simulink model "simulare1"  (R2026a)
settings: Solver=FixedStepAuto  StopTime=0.5  FixedStep=1e-6
values from neighbouring files (symbols this model uses):
  C = delta_I_l/(8*fs*delta_U_out)    (= 0.0021875)    [proiect.m]    (also in tema3.m = 0.0018)
  C_real = 1800e-6    (= 0.0018)    [proiect.m]
  L = (u_in - u_out)*mu/(fs*delta_I_l)    (= 0.00260416666667)    [proiect.m]    (also in tema3.m = 0.0025)
  L_real = 2.5e-3    (= 0.0025)    [proiect.m]
  mu = u_out/u_in    (= 0.416666666667)    [proiect.m]    (also in tema2_simscape.m; tema3_figuri.m = out.logsout.get('mu').Values)
  R = u_out/I_out_max    (= 1.25)    [proiect.m]    (also in tema2_simscape.m; tema3.m)
settings Model: Creator=Fer Alexandru  LastModifiedBy=Fer Alexandru

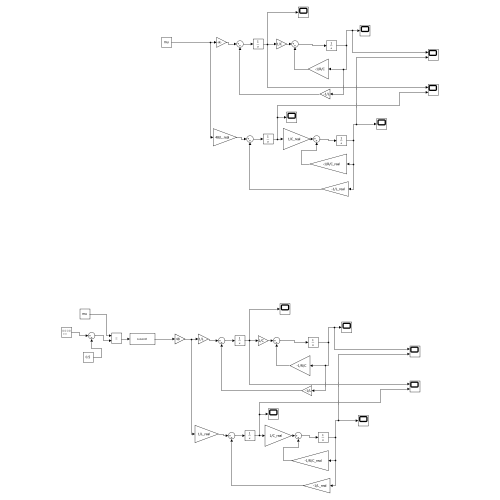
[thumbnail: Simulink's stored preview of the top-level diagram]
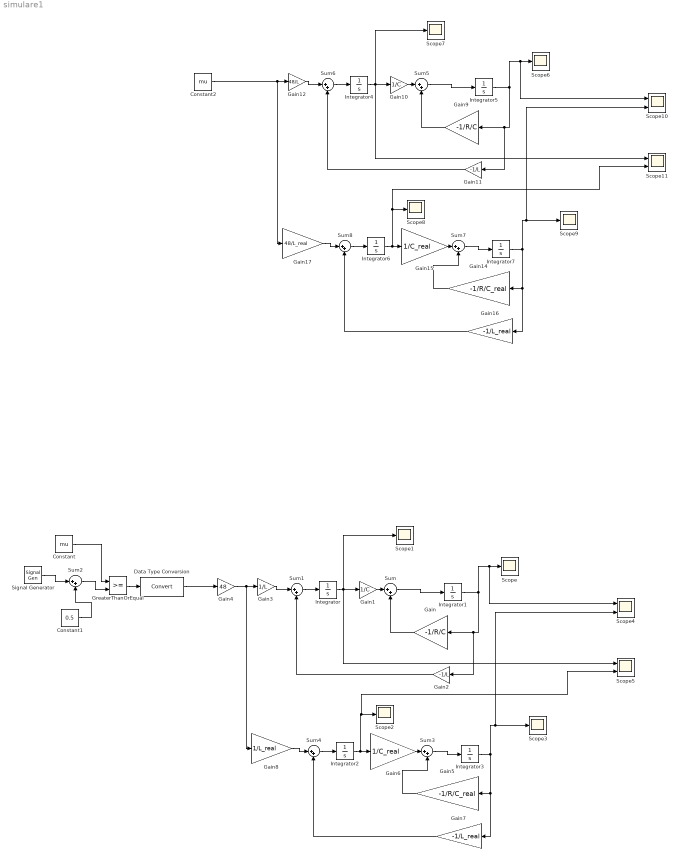
== system simulare1 ==
  Constant : Constant  Value=mu
  Constant1 : Constant  Value=0.5
  Constant2 : Constant  Value=mu
  Data Type Conversion : DataTypeConversion  SaturateOnIntegerOverflow=off  RndMeth=Floor
  Gain : Gain  Gain=-1/R/C
  Gain1 : Gain  Gain=1/C
  Gain10 : Gain  Gain=1/C
  Gain11 : Gain  Gain=-1/L
  Gain12 : Gain  Gain=48/L
  Gain14 : Gain  Gain=-1/R/C_real
  Gain15 : Gain  Gain=1/C_real
  Gain16 : Gain  Gain=-1/L_real
  Gain17 : Gain  Gain=48/L_real
  Gain2 : Gain  Gain=-1/L
  Gain3 : Gain  Gain=1/L
  Gain4 : Gain  Gain=48
  Gain5 : Gain  Gain=-1/R/C_real
  Gain6 : Gain  Gain=1/C_real
  Gain7 : Gain  Gain=-1/L_real
  Gain8 : Gain  Gain=1/L_real
  Gain9 : Gain  Gain=-1/R/C
  GreaterThanOrEqual : RelationalOperator  OutDataTypeStr=boolean  RndMeth=Simplest  InputSameDT=off
  Integrator{,1..7} (8 alike) : Integrator
  Scope{,1..3,6..9} (8 alike) : Scope
      Scope settings: ActiveDisplayYMinimum=19.471806262119504  ActiveDisplayYMaximum=19.914867992348224
      Scope1 settings: ActiveDisplayYMinimum=-2.4653855800406355  ActiveDisplayYMaximum=41.613009879574278
      Scope2 settings: ActiveDisplayYMinimum=38.565618567578547  ActiveDisplayYMaximum=49.041536557622351  DataLoggingVariableName=ScopeData2
      Scope3 settings: ActiveDisplayYMinimum=-12.707972209592477  ActiveDisplayYMaximum=48.224722703702227  DataLoggingVariableName=ScopeData3
      Scope6 settings: ActiveDisplayYMinimum=-11.374874550806879  ActiveDisplayYMaximum=44.740881240594341  DataLoggingVariableName=ScopeData8
      Scope7 settings: ActiveDisplayYMinimum=-9.753372524977701  ActiveDisplayYMaximum=69.089914194920084  DataLoggingVariableName=ScopeData9
      Scope8 settings: ActiveDisplayYMinimum=38.565618567578547  ActiveDisplayYMaximum=49.041536557622351  DataLoggingVariableName=ScopeData10
      Scope9 settings: ActiveDisplayYMinimum=-12.707972209592477  ActiveDisplayYMaximum=48.224722703702227  DataLoggingVariableName=ScopeData11
  Scope{4..5,10..11} (4 alike) : Scope  NumInputPorts=2
      Scope10 settings: ActiveDisplayYMinimum=19.282722022704462  ActiveDisplayYMaximum=20.523932646828097  DataLoggingVariableName=ScopeData6
      Scope11 settings: ActiveDisplayYMinimum=-115.01434593507554  ActiveDisplayYMaximum=164.705932550843  DataLoggingVariableName=ScopeData7
      Scope4 settings: ActiveDisplayYMinimum=19.282722022704462  ActiveDisplayYMaximum=20.523932646828097  DataLoggingVariableName=ScopeData4
      Scope5 settings: ActiveDisplayYMinimum=-115.01434593507554  ActiveDisplayYMaximum=164.705932550843  DataLoggingVariableName=ScopeData5
  Signal Generator : SignalGenerator  WaveForm=sawtooth  Amplitude=0.5  Frequency=800
  Sum{,1..8} (9 alike) : Sum  Inputs=|++
  wires:
  Integrator1/1 -> Gain2/1, Gain/1, Scope4/1, Scope/1
  Gain/1 -> Sum/2
  Integrator/1 -> Scope5/1, Scope1/1, Gain1/1
  Sum/1 -> Integrator1/1
  Gain1/1 -> Sum/1
  Gain2/1 -> Sum1/2
  Sum1/1 -> Integrator/1
  Signal Generator/1 -> Sum2/1
  Constant1/1 -> Sum2/2
  Sum2/1 -> GreaterThanOrEqual/2
  Constant/1 -> GreaterThanOrEqual/1
  GreaterThanOrEqual/1 -> Data Type Conversion/1
  Data Type Conversion/1 -> Gain4/1
  Gain3/1 -> Sum1/1
  Integrator3/1 -> Scope4/2, Scope3/1, Gain7/1, Gain5/1
  Gain7/1 -> Sum4/2
  Sum4/1 -> Integrator2/1
  Gain8/1 -> Sum4/1
  Gain4/1 -> Gain8/1, Gain3/1
  Gain5/1 -> Sum3/2
  Gain6/1 -> Sum3/1
  Integrator2/1 -> Scope5/2, Scope2/1, Gain6/1
  Sum3/1 -> Integrator3/1
  Gain14/1 -> Sum7/2
  Gain15/1 -> Sum7/1
  Gain17/1 -> Sum8/1
  Sum8/1 -> Integrator6/1
  Constant2/1 -> Gain17/1, Gain12/1
  Sum7/1 -> Integrator7/1
  Integrator6/1 -> Scope11/2, Scope8/1, Gain15/1
  Gain16/1 -> Sum8/2
  Integrator7/1 -> Scope10/2, Scope9/1, Gain16/1, Gain14/1
  Gain11/1 -> Sum6/2
  Integrator5/1 -> Gain11/1, Gain9/1, Scope10/1, Scope6/1
  Sum6/1 -> Integrator4/1
  Gain12/1 -> Sum6/1
  Gain9/1 -> Sum5/2
  Gain10/1 -> Sum5/1
  Integrator4/1 -> Scope11/1, Scope7/1, Gain10/1
  Sum5/1 -> Integrator5/1
